simulink model "SignalChainModelWithNCO"  (R2025b)
settings: Solver=FixedStepDiscrete  StartTime=0.0  StopTime=6000/Fs  RelTol=1e-3
undefined symbols (not defined in the file): Add, Fs, Shift
libraries: dsphdlmathfun2 x1, dsphdlxfrm2 x1, dsphdlsigops2 x1
settings Model: Creator=caleb  LastModifiedBy=caleb

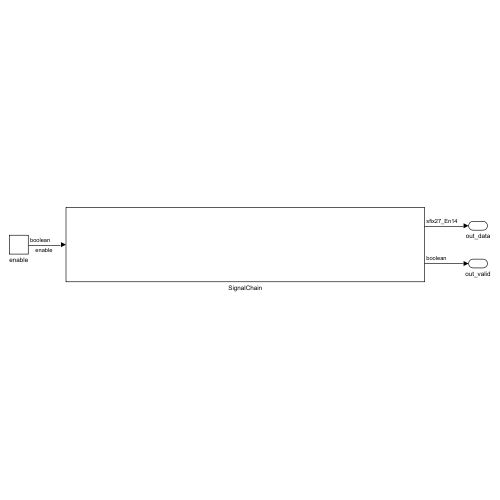
[thumbnail: Simulink's stored preview of the top-level diagram]
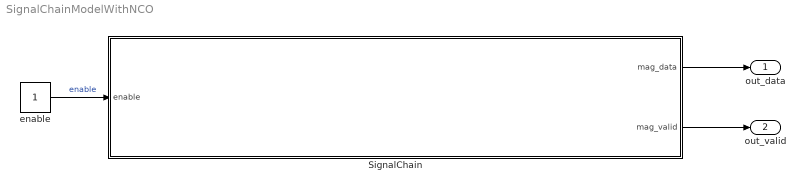
== system SignalChainModelWithNCO ==
  SignalChain : Subsystem  TreatAsAtomicUnit=on
  enable : Constant  OutDataTypeStr=boolean  SampleTime=1/Fs
  out_data : Outport  VectorParamsAs1DForOutWhenUnconnected=off
  out_valid : Outport  Port=2  VectorParamsAs1DForOutWhenUnconnected=off
  wires:
  enable/1 -> SignalChain/1(enable)  "enable"
  SignalChain/1(mag_data) -> out_data/1
  SignalChain/2(mag_valid) -> out_valid/1

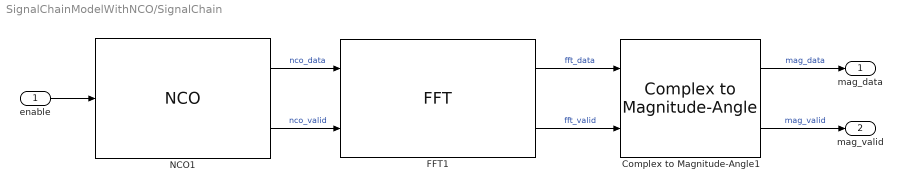
== system SignalChainModelWithNCO/SignalChain ==
  enable : Inport
  Complex to Magnitude-Angle1 : dsphdlmathfun2/Complex to Magnitude-Angle  NumIterationsSource=Auto  NumIterations=10  OutputFormat=Magnitude  AngleFormat=Normalized  ScaleOutput=on  ScalingMethod=Shift-Add  SimulateUsing=Code generation
  FFT1 : dsphdlxfrm2/FFT  Architecture=Streaming Radix 2^2  FFTLengthSource=Property  FFTLength=NFFT  FFTLengthMax=1024  ComplexMultiplication=Use 4 multipliers and 2 adders  BitReversedOutput=off  BitReversedInput=off  Normalize=off  SimulateUsing=Code generation  RoundingMethod=Floor  ResetInputPort=off  StartOutputPort=off  EndOutputPort=off
  NCO1 : dsphdlsigops2/NCO  PhaseIncrementSource=Property  PhaseIncrement=phase_increment  PhaseOffsetSource=Property  PhaseOffset=phase_offset  DitherSource=Property  NumDitherBits=dither_bits  SamplesPerFrame=1  LUTCompress=off  ResetAction=off  Waveform=Sine  PhasePort=off  SimulateUsing=Code generation  AccumulatorWL=16  PhaseQuantization=on  NumQuantizerAccumulatorBits=12  OutputDataType=Binary point scaling  OutputWL=16  OutputFL=14
      settings: LibrarySourceBlock=dsphdlsrcs2/NCO
  mag_data : Outport
  mag_valid : Outport  Port=2
  wires:
  Complex to Magnitude-Angle1/1 -> mag_data/1  "mag_data"
  NCO1/2 -> FFT1/2  "nco_valid"
  Complex to Magnitude-Angle1/2 -> mag_valid/1  "mag_valid"
  NCO1/1 -> FFT1/1  "nco_data"
  FFT1/1 -> Complex to Magnitude-Angle1/1  "fft_data"
  enable/1 -> NCO1/1
  FFT1/2 -> Complex to Magnitude-Angle1/2  "fft_valid"
